simulink model "exp3"  (R2023b)
settings: Solver=VariableStepAuto  StartTime=0.0  StopTime=1.5  RelTol=1e-3
libraries: spsDiodeLib x4, spsIGBTDiodeLib x4, spsSeriesRLCBranchLib x4, spsVoltageMeasurementLib x3, spsCurrentMeasurementLib x2, eePowerMeasurement x2, spsDCVoltageSourceLib x1, spsMutualInductanceLib x1, sps_lib x1
settings Model: Creator=manik  LastModifiedBy=muges

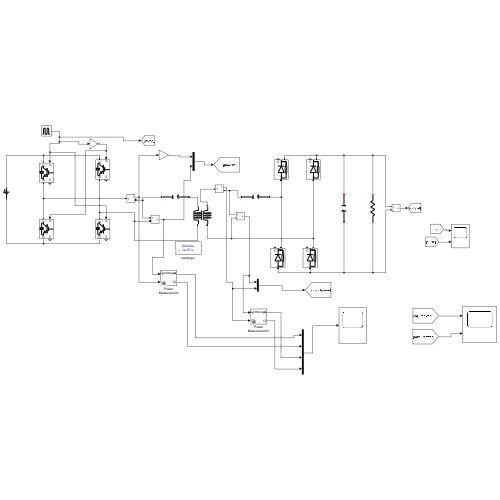
[thumbnail: Simulink's stored preview of the top-level diagram]
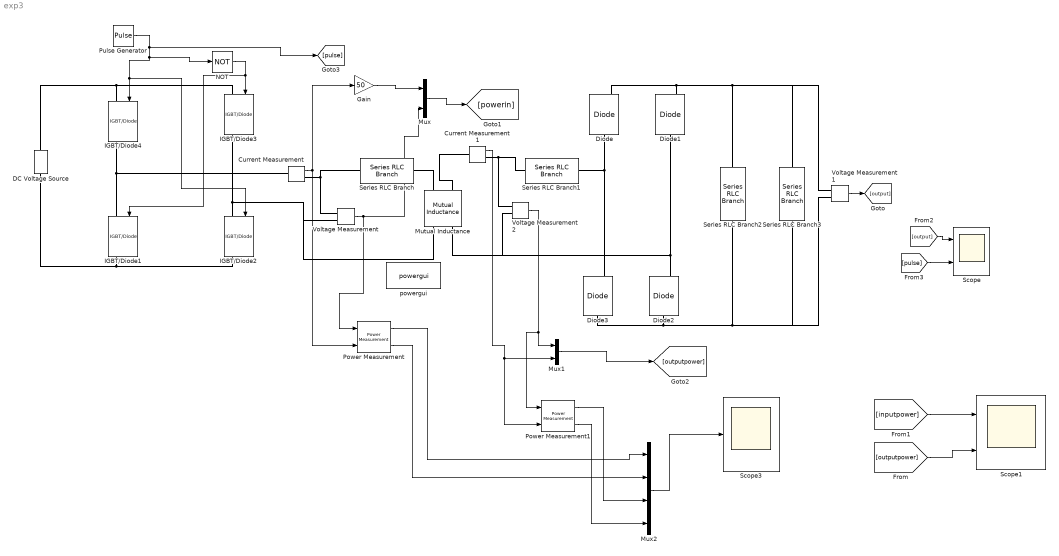
== system exp3 ==
  Current Measurement : spsCurrentMeasurementLib/Current Measurement  PhasorSimulation=off  OutputType=Complex  PSBequivalent=0
  Current Measurement1 : spsCurrentMeasurementLib/Current Measurement  PhasorSimulation=off  OutputType=Complex  PSBequivalent=0
  DC Voltage Source : spsDCVoltageSourceLib/DC Voltage Source  Amplitude=100  Measurements=None
  Diode{,1..3} (4 alike) : spsDiodeLib/Diode  Ron=0.001  Lon=0  Vf=0.8  IC=0  UseSnubber=0  Rs=500  Cs=250e-9  Measurements=on
  Gain : Gain  Gain=50
  IGBT/Diode{1..4} (4 alike) : spsIGBTDiodeLib/IGBT//Diode  Ron=1e-3  Rs=1e5  Cs=inf  Measurements=on
  Mutual Inductance : spsMutualInductanceLib/Mutual Inductance  LConnTagsString=a|b  RConnTagsString=A|B  TypeOfMutual=Generalized mutual inductance  NumberOfWindings=2  SelfImpedance1=[1.1 1.1e-03]  SelfImpedance2=[ 1.1 1.1e-03]  ThreeWindings=on  SelfImpedance3=[ 1.1 1.1e-03]  MutualImpedance=[1.0 1.0e-03]  InductanceMatrix=|  ResistanceMatrix=|  Measurements=None
      InductanceMatrix=|
      | [1e-3 0.9e-3;
      |  0.9e-3 1e-3] * 1e-3
      ResistanceMatrix=|
      | [1 0;
      |  0 1]
      settings: LibrarySourceBlock=sps_lib/Passives/Mutual Inductance
  Mux : Mux  Inputs=2
  Mux1 : Mux  Inputs=2
  Mux2 : Mux
  NOT : Logic  Operator=NOT  IconShape=distinctive  AllPortsSameDT=off  OutDataTypeStr=boolean
  Power Measurement : eePowerMeasurement/Power Measurement  LabelModeActiveChoice=Continuous  F=60  K=[0 1 2 3]  Ts=0
  Power Measurement1 : eePowerMeasurement/Power Measurement  LabelModeActiveChoice=Continuous  F=60  K=[0 1 2 3]  Ts=0
  Pulse Generator : DiscretePulseGenerator  PulseType=Time based  Period=10  PulseWidth=5
  Scope : Scope  NumInputPorts=2
  Scope1 : Scope  NumInputPorts=2
  Scope3 : Scope
  Series RLC Branch : spsSeriesRLCBranchLib/Series RLC Branch  LConnTagsString=__new0  RConnTagsString=__new0  BranchType=C  Resistance=1  Inductance=1e-3  SetiL0=off  InitialCurrent=0  Capacitance=1.0132e-08  Setx0=off  InitialVoltage=0  Measurements=None
  Series RLC Branch1 : spsSeriesRLCBranchLib/Series RLC Branch  LConnTagsString=__new0  RConnTagsString=__new0  BranchType=C  Resistance=1  Inductance=1e-3  SetiL0=off  InitialCurrent=0  Capacitance=1.0132e-08  Setx0=off  InitialVoltage=0  Measurements=None
  Series RLC Branch2 : spsSeriesRLCBranchLib/Series RLC Branch  LConnTagsString=__new0  RConnTagsString=__new0  BranchType=C  Resistance=1  Inductance=1e-3  SetiL0=off  InitialCurrent=0  Capacitance=220e-06  Setx0=off  InitialVoltage=0  Measurements=None
  Series RLC Branch3 : spsSeriesRLCBranchLib/Series RLC Branch  LConnTagsString=__new0  RConnTagsString=__new0  BranchType=R  Resistance=100  Inductance=1e-3  SetiL0=off  InitialCurrent=0  Capacitance=1.0132e-08  Setx0=off  InitialVoltage=0  Measurements=None
  Voltage Measurement : spsVoltageMeasurementLib/Voltage Measurement  PhasorSimulation=off  OutputType=Complex  PSBequivalent=0
  Voltage Measurement1 : spsVoltageMeasurementLib/Voltage Measurement  PhasorSimulation=off  OutputType=Complex  PSBequivalent=0
  Voltage Measurement2 : spsVoltageMeasurementLib/Voltage Measurement  PhasorSimulation=off  OutputType=Complex  PSBequivalent=0
  powergui : sps_lib/powergui  Priority=1  SimulationMode=Discrete  SampleTime=1e-07  frequency=60  Iterations=50  frequencyindice=0  Pbase=100e6  ErrMax=1e-4  UnitsV=kV  UnitsW=MW  buscounter=0  FunctionMessages=off  echomessages=off  EnableUseOfTLC=off  CurrentSourceSwitches=off  DisableSnubberDevices=off  DisableRonSwitches=off  DisableVfSwitches=off  DisplayEquations=off  AutomaticDiscreteSolvers=off  SolverType=Tustin/Backward Euler (TBE)  Interpol=off  ExternalGateDelay=off  methode=off  Ts=100  x0status=blocks  SPID=on  SwTol=0  HookPort=off  NonlinearTolerance=1e-4  nMaxIteration=100  ContinueOnMaxIteration=off  RestoreLinks=warning  ResistiveCurrentMeasurement=off  Frange=[0:2:500]  Ylog=off  Xlog=on  ShowGrid=off  save=off  variable=ZData  structure=0  ZoomFFT=off  StartTime=0.0  cycles=1  DisplayStyle=1  fundamental=60  FreqAxis=off  MaxFrequency=1000  frequencyindicesteady=1  RmsSteady=1  display=off
  wires:
  Current Measurement/1 -> Gain/1, Power Measurement/2
  Gain/1 -> Mux/1
  Voltage Measurement/1 -> Power Measurement/1, Mux/2
  Voltage Measurement2/1 -> Power Measurement1/1, Mux1/1
  Current Measurement1/1 -> Power Measurement1/2, Mux1/2
  Mux1/1 -> [outputpower]
  Mux2/1 -> Scope3/1
  Power Measurement/1 -> Mux2/1
  Power Measurement/2 -> Mux2/2
  Power Measurement1/1 -> Mux2/3
  Power Measurement1/2 -> Mux2/4
  Pulse Generator/1 -> [pulse], NOT/1, IGBT/Diode2/1, IGBT/Diode4/1
  NOT/1 -> IGBT/Diode1/1, IGBT/Diode3/1
  Voltage Measurement1/1 -> [output]
  Mux/1 -> [powerin]
  [outputpower] -> Scope1/2
  [inputpower] -> Scope1/1
  [output] -> Scope/1
  [pulse] -> Scope/2
  connections:
  Current Measurement/LConn1 -- IGBT/Diode4/RConn1 -- IGBT/Diode1/LConn1
  IGBT/Diode1/RConn1 -- DC Voltage Source/LConn1 -- IGBT/Diode2/RConn1
  IGBT/Diode3/RConn1 -- Mutual Inductance/RConn1 -- Voltage Measurement/LConn2 -- IGBT/Diode2/LConn1
  IGBT/Diode3/LConn1 -- IGBT/Diode4/LConn1 -- DC Voltage Source/RConn1
  Series RLC Branch/LConn1 -- Voltage Measurement/LConn1 -- Current Measurement/RConn1
  Series RLC Branch/RConn1 -- Mutual Inductance/LConn1
  Diode3/RConn1 -- Series RLC Branch1/RConn1 -- Diode/LConn1
  Diode1/LConn1 -- Voltage Measurement2/LConn2 -- Mutual Inductance/RConn2 -- Diode2/RConn1
  Series RLC Branch2/RConn1 -- Series RLC Branch3/RConn1 -- Voltage Measurement1/LConn2 -- Diode2/LConn1 -- Diode3/LConn1
  Diode/RConn1 -- Series RLC Branch3/LConn1 -- Voltage Measurement1/LConn1 -- Series RLC Branch2/LConn1 -- Diode1/RConn1
  Mutual Inductance/LConn2 -- Current Measurement1/LConn1
  Series RLC Branch1/LConn1 -- Voltage Measurement2/LConn1 -- Current Measurement1/RConn1
